simulink model "b0_foc2"  (R2023b)
settings: Solver=FixedStepDiscrete  StartTime=0.0  StopTime=150  FixedStep=0.001  RelTol=1e-3
undefined symbols (not defined in the file or in its folder): DiscIntNeverNeededParam
settings Model: Creator=28447  LastModifiedBy=28447
settings SFSimCC: SimUserIncludeDirs=D:\Desktop\RCESO\simulink
settings SFSimCC: SimCustomHeaderCode=|
  | typedef struct { float b0; float du; } b0_res_t;
  | extern b0_res_t b0_ident_res(float iq, float u, float omega, float e1, float v);
settings SFSimCC: SimUserSources=|
  | D:\Desktop\RCESO\simulink\b0_ident.c
  | D:\Desktop\RCESO\simulink\b0_ident_wrap.c

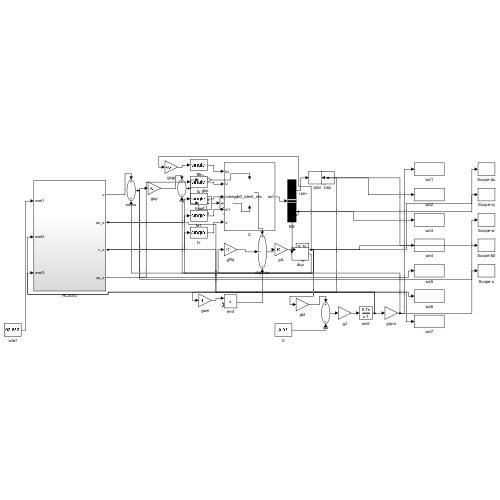
[thumbnail: Simulink's stored preview of the top-level diagram]
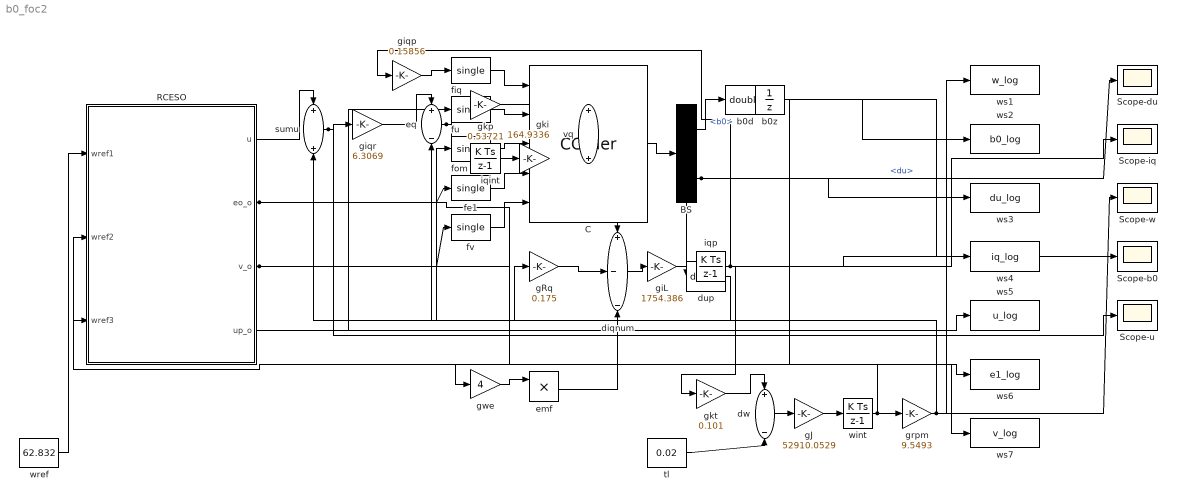
== system b0_foc2 ==
  BS : BusSelector  OutputSignals=b0,du
  C : CCaller  FunctionName=b0_ident_res  PortSpecificationStruct="%)30     .    4 H   8    (     @         %    \"     8    !     0         %  0 \"0    $    _    07)G3F%M90  4&]R=$YA;64 4V-O<&4     26YD97@     5'EP90      4VEZ90      27-';&]B86P   X    P    !@    @    $          4    (     0    ,    !         !   P!O=70 #@   #     &    \"     0         !0    @    !     P    $         $  # &]U=  .    .     8    (    !          %    \"     $    &     0         0   ...(+3175 chars)"
  RCESO : Subsystem
  Scope-b0 : Scope
  Scope-du : Scope
  Scope-iq : Scope
  Scope-u : Scope
  Scope-w : Scope
  b0d : DataTypeConversion  OutDataTypeStr=double  SaturateOnIntegerOverflow=off  RndMeth=Floor
  b0z : UnitDelay  InitialCondition=400  SampleTime=0.001  HasFrameUpgradeWarning=on
  diqnum : Sum  Inputs=+--
  dup : DataTypeConversion  OutDataTypeStr=double  SaturateOnIntegerOverflow=off  RndMeth=Floor
  dw : Sum  Inputs=+-
  emf : Product
  eq : Sum  Inputs=+-
  fe1 : DataTypeConversion  OutDataTypeStr=single  SaturateOnIntegerOverflow=off  RndMeth=Floor
  fiq : DataTypeConversion  OutDataTypeStr=single  SaturateOnIntegerOverflow=off  RndMeth=Floor
  fom : DataTypeConversion  OutDataTypeStr=single  SaturateOnIntegerOverflow=off  RndMeth=Floor
  fu : DataTypeConversion  OutDataTypeStr=single  SaturateOnIntegerOverflow=off  RndMeth=Floor
  fv : DataTypeConversion  OutDataTypeStr=single  SaturateOnIntegerOverflow=off  RndMeth=Floor
  gJ : Gain  Gain=52910.0529
  gRq : Gain  Gain=0.175
  giL : Gain  Gain=1754.386
  giqp : Gain  Gain=0.15856
  giqr : Gain  Gain=6.3069
  gki : Gain  Gain=164.9336
  gkp : Gain  Gain=0.53721
  gkt : Gain  Gain=0.101
  grpm : Gain  Gain=9.5493
  gwe : Gain  Gain=4
  iqint : DiscreteIntegrator  SampleTime=0.001  ICPrevOutput=DiscIntNeverNeededParam  ICPrevScaledInput=DiscIntNeverNeededParam
  iqp : DiscreteIntegrator  SampleTime=0.001  ICPrevOutput=DiscIntNeverNeededParam  ICPrevScaledInput=DiscIntNeverNeededParam
  sumu : Sum
  tl : Constant  Value=0.02  SampleTime=0.001
  vq : Sum
  wint : DiscreteIntegrator  SampleTime=0.001  ICPrevOutput=DiscIntNeverNeededParam  ICPrevScaledInput=DiscIntNeverNeededParam
  wref : Constant  Value=62.832  SampleTime=0.001
  ws1 : ToWorkspace  VariableName=w_log  SaveFormat=Timeseries  SampleTime=0.001
  ws2 : ToWorkspace  VariableName=b0_log  SaveFormat=Timeseries  SampleTime=0.001
  ws3 : ToWorkspace  VariableName=du_log  SaveFormat=Timeseries  SampleTime=0.001
  ws4 : ToWorkspace  VariableName=iq_log  SaveFormat=Timeseries  SampleTime=0.001
  ws5 : ToWorkspace  VariableName=u_log  SaveFormat=Timeseries  SampleTime=0.001
  ws6 : ToWorkspace  VariableName=e1_log  SaveFormat=Timeseries  SampleTime=0.001
  ws7 : ToWorkspace  VariableName=v_log  SaveFormat=Timeseries  SampleTime=0.001
  wires:
  giqp/1 -> fiq/1
  fiq/1 -> C/1
  RCESO/4(up_o) -> fu/1
  fu/1 -> C/2
  grpm/1 -> fom/1, ws1/1, Scope-w/1
  fom/1 -> C/3
  RCESO/2(eo_o) -> fe1/1, ws6/1
  fe1/1 -> C/4
  RCESO/3(v_o) -> fv/1, ws7/1
  fv/1 -> C/5
  C/1 -> BS/1
  BS/1 -> b0d/1  "<b0>"
  b0d/1 -> b0z/1, ws2/1, Scope-b0/1
  BS/2 -> dup/1, ws3/1, Scope-du/1  "<du>"
  RCESO/1(u) -> sumu/1
  dup/1 -> sumu/2
  wref/1 -> RCESO/1(wref1)
  wint/1 -> RCESO/2(wref2), gwe/1, grpm/1
  b0z/1 -> RCESO/3(wref3)
  sumu/1 -> giqr/1, ws5/1, Scope-u/1
  giqr/1 -> eq/1
  iqp/1 -> eq/2, gRq/1, gkt/1, giqp/1, ws4/1, Scope-iq/1
  eq/1 -> gkp/1, iqint/1
  iqint/1 -> gki/1
  gkp/1 -> vq/1
  gki/1 -> vq/2
  vq/1 -> diqnum/1
  gRq/1 -> diqnum/2
  emf/1 -> diqnum/3
  diqnum/1 -> giL/1
  giL/1 -> iqp/1
  gwe/1 -> emf/1
  gkt/1 -> dw/1
  tl/1 -> dw/2
  dw/1 -> gJ/1
  gJ/1 -> wint/1

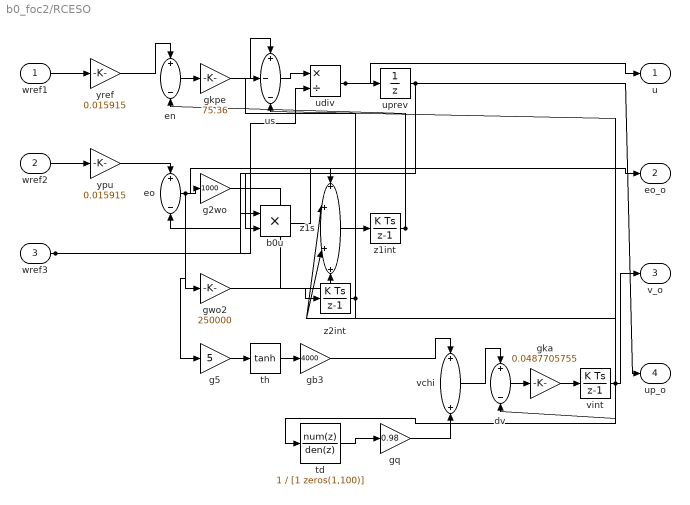
== system b0_foc2/RCESO ==
  wref1 : Inport
  wref2 : Inport  Port=2
  wref3 : Inport  Port=3
  b0u : Product
  dv : Sum  Inputs=+-
  en : Sum  Inputs=+-
  eo : Sum  Inputs=+-
  g2wo : Gain  Gain=1000
  g5 : Gain  Gain=5
  gb3 : Gain  Gain=4000
  gka : Gain  Gain=0.0487705755
  gkpe : Gain  Gain=75.36
  gq : Gain  Gain=0.98
  gwo2 : Gain  Gain=250000
  td : DiscreteTransferFcn  Numerator=1  Denominator=[1 zeros(1,100)]  SampleTime=0.001
  th : Trigonometry  Operator=tanh
  udiv : Product  Inputs=*/
  uprev : UnitDelay  SampleTime=0.001  HasFrameUpgradeWarning=on
  us : Sum  Inputs=+--
  vchi : Sum
  vint : DiscreteIntegrator  SampleTime=0.001  ICPrevOutput=DiscIntNeverNeededParam  ICPrevScaledInput=DiscIntNeverNeededParam
  ypu : Gain  Gain=0.015915
  yref : Gain  Gain=0.015915
  z1int : DiscreteIntegrator  SampleTime=0.001  ICPrevOutput=DiscIntNeverNeededParam  ICPrevScaledInput=DiscIntNeverNeededParam
  z1s : Sum  Inputs=++++
  z2int : DiscreteIntegrator  SampleTime=0.001  ICPrevOutput=DiscIntNeverNeededParam  ICPrevScaledInput=DiscIntNeverNeededParam
  u : Outport
  eo_o : Outport  Port=2
  v_o : Outport  Port=3
  up_o : Outport  Port=4
  wires:
  ? -> ?
  wref1/1 -> yref/1
  wref2/1 -> ypu/1
  yref/1 -> en/1
  z1int/1 -> en/2, eo/2
  en/1 -> gkpe/1
  gkpe/1 -> us/1
  z2int/1 -> us/2, z1s/3
  vint/1 -> us/3, z1s/2, td/1, dv/2, v_o/1
  us/1 -> udiv/1
  wref3/1 -> udiv/2, b0u/1
  udiv/1 -> u/1, uprev/1
  uprev/1 -> up_o/1, b0u/2
  ypu/1 -> eo/1
  eo/1 -> eo_o/1, g2wo/1, gwo2/1, g5/1
  g2wo/1 -> z1s/4
  b0u/1 -> z1s/1
  z1s/1 -> z1int/1
  gwo2/1 -> z2int/1
  g5/1 -> th/1
  th/1 -> gb3/1
  td/1 -> gq/1
  gb3/1 -> vchi/1
  gq/1 -> vchi/2
  vchi/1 -> dv/1
  dv/1 -> gka/1
  gka/1 -> vint/1
